simulink model "proof_of_concept"  (R2026a)
settings: Solver=ode4  StopTime=120  FixedStep=0.002
undefined symbols (not defined in the file or in its folder): IC0
libraries: simulink x1
settings Model: Creator=aayush  LastModifiedBy=aayush

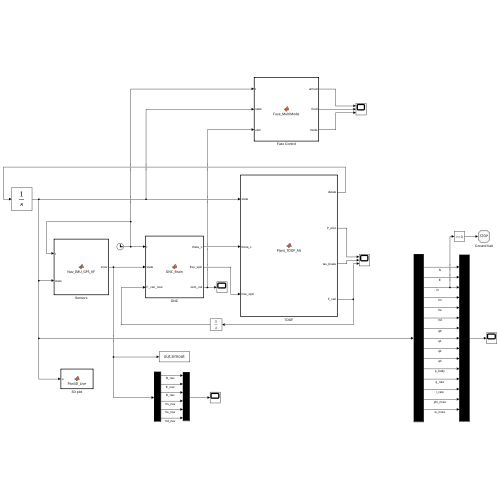
[thumbnail: Simulink's stored preview of the top-level diagram]
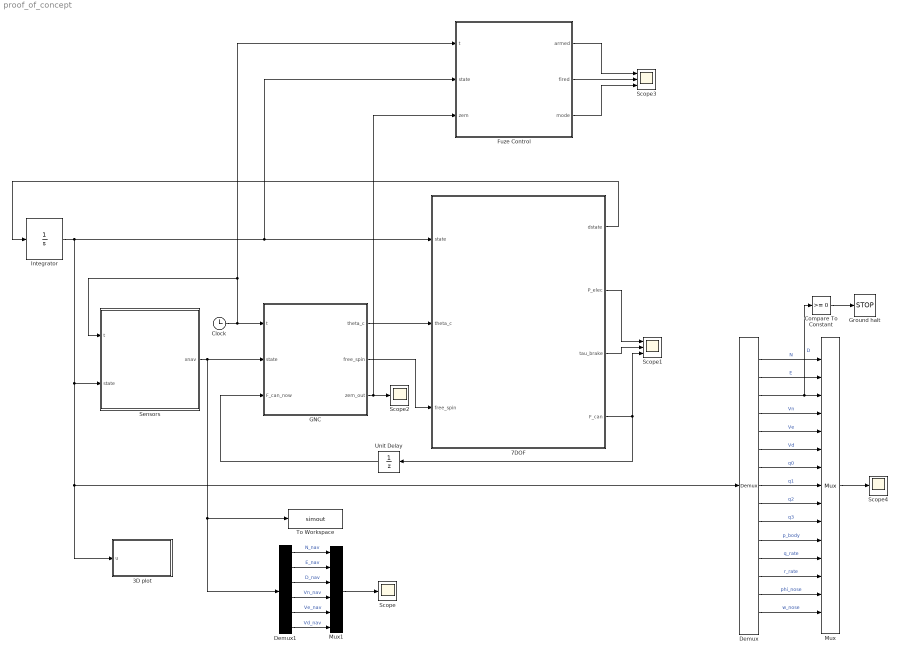
== system proof_of_concept ==
  3D plot : MATLAB Function  TreatAsAtomicUnit=on
  7DOF : MATLAB Function  TreatAsAtomicUnit=on
  Clock : Clock
  Compare To Constant : simulink/Logic and Bit Operations/Compare To Constant  relop=>=  const=0  OutDataTypeStr=boolean
  Demux : Demux  Outputs=15
  Demux1 : Demux  Outputs=6
  Fuze Control : MATLAB Function  TreatAsAtomicUnit=on
  GNC : MATLAB Function  TreatAsAtomicUnit=on
  Ground halt : Stop
  Integrator : Integrator  InitialCondition=IC0
  Mux : Mux  Inputs=15
  Mux1 : Mux  Inputs=6
  Scope : Scope
      settings: ActiveDisplayYMinimum=-6497.6621152905909  ActiveDisplayYMaximum=23835.158611575058
  Scope1 : Scope  NumInputPorts=3
      settings: ActiveDisplayYMinimum=-36.379053196985673  ActiveDisplayYMaximum=247.41147877287113
  Scope2 : Scope
      settings: ActiveDisplayYMinimum=-412.03643421286256  ActiveDisplayYMaximum=3708.3279079157642  DataLoggingVariableName=ScopeData2
  Scope3 : Scope  NumInputPorts=3
      settings: ActiveDisplayYMinimum=-0.12499999999999997  ActiveDisplayYMaximum=1.125  DataLoggingVariableName=ScopeData3
  Scope4 : Scope
      settings: ActiveDisplayYMinimum=-6498.1534286877359  ActiveDisplayYMaximum=23841.089492594823  DataLoggingVariableName=ScopeData4
  Sensors : MATLAB Function  TreatAsAtomicUnit=on
  To Workspace : ToWorkspace  VariableName=simout  SaveFormat=Timeseries  SampleTime=-1
  Unit Delay : UnitDelay  SampleTime=-1
  wires:
  GNC/1(theta_c) -> 7DOF/2(theta_c)
  GNC/2(free_spin) -> 7DOF/3(free_spin)
  7DOF/1(dstate) -> Integrator/1
  Clock/1 -> GNC/1(t), Fuze Control/1(t), Sensors/1(t)
  Integrator/1 -> Demux/1, 3D plot/1(u), Sensors/2(state), Fuze Control/2(state), 7DOF/1(state)
  7DOF/3(tau_brake) -> Scope1/2
  7DOF/2(P_elec) -> Scope1/1
  7DOF/4(F_can) -> Unit Delay/1, Scope1/3
  GNC/3(zem_out) -> Fuze Control/3(zem), Scope2/1
  Unit Delay/1 -> GNC/3(F_can_now)
  Sensors/1(xnav) -> Demux1/1, To Workspace/1, GNC/2(state)
  Fuze Control/2(fired) -> Scope3/2
  Fuze Control/1(armed) -> Scope3/1
  Fuze Control/3(mode) -> Scope3/3
  Demux/1 -> Mux/1  "N"
  Demux/2 -> Mux/2  "E"
  Demux/3 -> Compare To Constant/1, Mux/3  "D"
  Demux/4 -> Mux/4  "Vn"
  Demux/5 -> Mux/5  "Ve"
  Demux/6 -> Mux/6  "Vd"
  Demux/7 -> Mux/7  "q0"
  Demux/8 -> Mux/8  "q1"
  Demux/9 -> Mux/9  "q2"
  Demux/10 -> Mux/10  "q3"
  Demux/11 -> Mux/11  "p_body"
  Demux/12 -> Mux/12  "q_rate"
  Demux/13 -> Mux/13  "r_rate"
  Demux/14 -> Mux/14  "phi_nose"
  Demux/15 -> Mux/15  "w_nose"
  Demux1/3 -> Mux1/3  "D_nav"
  Demux1/1 -> Mux1/1  "N_nav"
  Demux1/2 -> Mux1/2  "E_nav"
  Demux1/4 -> Mux1/4  "Vn_nav"
  Demux1/5 -> Mux1/5  "Ve_nav"
  Demux1/6 -> Mux1/6  "Vd_nav"
  Mux1/1 -> Scope/1
  Mux/1 -> Scope4/1
  Compare To Constant/1 -> Ground halt/1

== matlab function proof_of_concept/GNC ==
  settings: updateMethod=DISCRETE
  data: t input; theta_c output; state input; free_spin output; zem_out output; F_can_now input
function [theta_c, free_spin, zem_out] = GNC_Brain(t, state, F_can_now)
    persistent th_c fs last_F tgt_xy locked mode_free checked failsafe next_ctrl zem_p
    if isempty(th_c) || t < 0.05
        th_c = 0; fs = true; last_F = 0; tgt_xy = [0;0];
        locked = false; mode_free = true; checked = false;
        failsafe = false; next_ctrl = 0; zem_p = 0;
    end
    last_F = 0.65*last_F + 0.35*F_can_now;
    theta_c = th_c; free_spin = fs; zem_out = zem_p;
    if t < next_ctrl, return; end
    next_ctrl = t + 0.02;

    Om_E  = 7.292115e-5*[cos(32*pi/180); 0; -sin(32*pi/180)];
    Mg    = [0.5 0.8 0.95 1.05 1.2 1.5 2.0 2.5];
    Cdrow = [0.13 0.145 0.24 0.30 0.255 0.20 0.18 0.17];

    r = state(1:3); v = state(4:6);
    sp0 = norm(v); if sp0 < 1.0, sp0 = 1.0; end
    vhat0 = v/sp0;
    des = [cos(th_c); sin(th_c); 0];
    fd = des - dot(des,vhat0)*vhat0;
    nfd = norm(fd); if nfd > 1e-6, fd = fd/nfd; else fd = [0;0;0]; end
    F_vec = last_F * fd;

    rr = r; vv = v; tp = 0;
    while rr(3) < 0 && tp < 70
        sp = norm(vv); if sp < 1.0, sp = 1.0; end
        h = max(-rr(3), 0);
        T = max(288.15 - 0.0065*h, 210.0);
        rho = 1.225*(T/288.15)^4.2559;
        Cd0 = lut(sp/sqrt(1.4*287.05*T), Mg, Cdrow);
        a = -Cd0*(0.5*rho*sp^2)*0.01887/43.5*(vv/sp) + F_vec/43.5 ...
            + [0;0;9.80665*(6371000/(6371000+h))^2] - 2*cross(Om_E, vv);
        vv = vv + a*0.1;
        rr = rr + vv*0.1;
        tp = tp + 0.1;
    end

    arm_time = 7.0; deadband = 0.0;    % PoC: hold to impact (no coast switch)
    if ~locked && t >= arm_time
        imp0 = predict0(r, v);
        tgt_xy = imp0(1:2) + [100; -70];
        locked = true;
    end

    if t < arm_time || failsafe
        fs = true; zem_p = 0;
    else
        zem_vec = tgt_xy - rr(1:2);
        zem = norm(zem_vec);
        zem_p = zem; zem_out = zem;
        if ~checked && t >= 8.0
            checked = true;
            if zem > 20000.0, failsafe = true; end
        end
        if ~failsafe
            if mode_free
                if zem >= 1.5*deadband, mode_free = false; end
            else
                if zem < deadband, mode_free = true; end
            end
        end
        fs = mode_free || failsafe;
        if ~fs
            desired = atan2(zem_vec(2), zem_vec(1));
            err = wrapPi(desired - th_c);
            rate = max(min(6.0*err, 1.5708), -1.5708);
            th_c = th_c + (0.02/(0.25+0.02))*rate*0.25;
        end
    end
    theta_c = th_c; free_spin = fs;
end

function imp = predict0(r, v)
    Om_E  = 7.292115e-5*[cos(32*pi/180); 0; -sin(32*pi/180)];
    Mg    = [0.5 0.8 0.95 1.05 1.2 1.5 2.0 2.5];
    Cdrow = [0.13 0.145 0.24 0.30 0.255 0.20 0.18 0.17];
    rr = r; vv = v; tp = 0;
    while rr(3) < 0 && tp < 70
        sp = norm(vv); if sp < 1.0, sp = 1.0; end
        h = max(-rr(3), 0);
        T = max(288.15 - 0.0065*h, 210.0);
        rho = 1.225*(T/288.15)^4.2559;
        Cd0 = lut(sp/sqrt(1.4*287.05*T), Mg, Cdrow);
        a = -Cd0*(0.5*rho*sp^2)*0.01887/43.5*(vv/sp) ...
            + [0;0;9.80665*(6371000/(6371000+h))^2] - 2*cross(Om_E, vv);
        vv = vv + a*0.1;
        rr = rr + vv*0.1;
        tp = tp + 0.1;
    end
    imp = [rr(1); rr(2); 0];
end

function y = lut(M, Mg, Vg)
    n = numel(Mg);
    if M <= Mg(1), y = Vg(1); return; end
    if M >= Mg(n), y = Vg(n); return; end
    k = 1;
    while k < n-1 && M > Mg(k+1), k = k+1; end
    y = Vg(k) + (M-Mg(k))/(Mg(k+1)-Mg(k)) * (Vg(k+1)-Vg(k));
end
function y = wrapPi(x)
    y = mod(x + pi, 2*pi) - pi;
end

== matlab function proof_of_concept/7DOF ==
  data: state input; dstate output; theta_c input; free_spin input; P_elec output; tau_brake output; F_can output
function [dstate, P_elec, tau_brake, F_can] = Plant_7DOF_Alt(state, theta_c, free_spin)
    r = state(1:3); v = state(4:6); q = state(7:10);
    w_b = state(11:13); phi_n = state(14); w_n = state(15);

    m = 43.5; Ixx = 0.148; Iyy = 1.82; Izz = 1.82; Ixx_n = 0.012;
    S = 0.01887; d = 0.155; r_c = 0.48;
    lat = 32*pi/180; Re = 6371000;
    Om_E = 7.292115e-5*[cos(lat); 0; -sin(lat)];

    h = max(-r(3), 0);
    T = max(288.15 - 0.0065*h, 210.0);
    rho = 1.225*(T/288.15)^4.2559;
    a_snd = sqrt(1.4*287.05*T);
    g_mag = 9.80665*(Re/(Re+h))^2;

    speed = norm(v); if speed < 1.0, speed = 1.0; end
    vhat = v/speed;
    M = speed/a_snd;
    qdyn = 0.5*rho*speed^2;

    % ===== Aero LUT (calibrated row; IDENTICAL in GNC predictors) =====
    Mg = [0.5 0.8 0.95 1.05 1.2 1.5 2.0 2.5];
    Cd0  = lut(M, Mg, [0.13 0.145 0.24 0.30 0.255 0.20 0.18 0.17]);
    Cl_a = lut(M, Mg, [1.70 1.68 1.55 1.45 1.50 1.55 1.50 1.45]);
    Cm_a = lut(M, Mg, [-2.4 -2.35 -2.1 -1.95 -2.15 -2.3 -2.25 -2.2]);
    Clp  = lut(M, Mg, [-0.04 -0.042 -0.05 -0.055 -0.05 -0.048 -0.045 -0.043]);
    Cmq  = lut(M, Mg, [-3.8 -4.0 -4.5 -4.6 -4.3 -4.1 -4.0 -3.9]);
    Cn_pa= lut(M, Mg, [0.04 0.05 0.07 0.08 0.06 0.05 0.04 0.035]);
    Cm_pa= lut(M, Mg, [-0.003 -0.0035 -0.005 -0.0055 -0.0045 -0.004 -0.0035 -0.003]);

    R = q_to_dcm(q); body_x = R(:,1);
    ca = max(min(dot(body_x, vhat),1),-1); aoa = acos(ca);
    F_drag = -Cd0*qdyn*S*vhat;
    F_lift = [0;0;0]; F_mag = [0;0;0]; M_im = [0;0;0];
    if aoa > 1e-4 && speed > 35
        ldir = (body_x - ca*vhat); ldir = ldir/norm(ldir);
        if free_spin
            Cl = 0.0;                              % rotating canards: net lift = 0
        else
            Cl = max(min(Cl_a*aoa, 1.05), -1.05);  % maneuvering: follow LUT
        end
        F_lift = Cl*qdyn*S*ldir;
        F_drag = F_drag - (Cl^2/(pi*0.75*5.2))*qdyn*S*vhat;
        axis2 = cross(body_x, vhat); axis2 = axis2/norm(axis2);
        pbar = w_b(1)*d/(2*speed);
        M_im = (-Cm_a*qdyn*S*d*aoa)*axis2 + (Cm_pa*qdyn*S*d*pbar*aoa)*axis2;
        F_mag = (Cn_pa*qdyn*S*pbar*aoa)*axis2;
    end

    % ===== Canards (hold/maneuver only, 3-D perpendicular force) =====
    F_can = [0;0;0];
    if ~free_spin && speed > 70 && abs(w_n) < 40
        CN0 = 1.0*0.68*0.00075/S;
        a_deg = aoa*180/pi;
        f_alpha = max(min(0.88 + 0.012*a_deg - 0.00015*a_deg^2, 1.25), 0.85);
        if aoa >= 0.95*(16*pi/180), f_alpha = f_alpha*0.7; end
        if M < 0.7, f_mach = 1.0;
        elseif M < 1.1, f_mach = 1.0 - 0.15*(M-0.7)/0.4;
        else, f_mach = 0.82; end
        f_mach = max(min(f_mach, 1.05), 0.75);
        f_spin = max(min(1.0 - (w_n/40.0)^2, 1.0), 0.0);
        cy = CN0*f_alpha*f_mach*f_spin;
        Fmag = min(cy*qdyn*S, 1.05*m);
        desired = [cos(phi_n); sin(phi_n); 0];
        f_dir = desired - dot(desired, vhat)*vhat;
        nrm = norm(f_dir);
        if nrm > 1e-6
            F_can = (Fmag/nrm)*f_dir;
            F_lift = F_lift*(1.0 - 0.15*min(Fmag/(qdyn*S), 1.0));
            F_drag = F_drag - 0.05*(Fmag/(qdyn*S))^2*qdyn*S*vhat;
        end
    end
    F_total = F_drag + F_lift + F_can + F_mag;

    kd = qdyn*S*d*(d/(2*speed));
    M_damp = [Clp*kd*w_b(1); Cmq*kd*w_b(2); Cmq*kd*w_b(3)];
    M_can = cross([r_c;0;0], R'*F_can);
    M_body = M_can + M_damp + R'*M_im;

    % ===== Dual-spin brake + alternator =====
    w_rel = w_n - w_b(1);
    tau_aero = 0.0;
    if speed > 40
        tau_aero = -0.00040*qdyn*sign(w_n)*min(abs(w_n)/80.0, 1.0);
        if abs(w_n) < 6.0, tau_aero = tau_aero*0.2; end
    end
    tau_alt = -0.00025*w_rel;
    if free_spin
        tau_cmd = tau_aero + tau_alt;
    else
        err_phi = wrapPi(theta_c - phi_n);
        tau_cmd = 0.15*tau_aero + tau_alt - 1.0*w_n + 30.0*err_phi;
    end
    tau_brake = max(min(tau_cmd, 8.0), -8.0) - 0.0015*w_rel;
    M_body(1) = M_body(1) - tau_brake;

    P_elec = 0.65*(1 - exp(-abs(w_rel)/200))*abs(tau_alt*w_rel);

    wdot = [ (M_body(1) - (Iyy-Izz)*w_b(2)*w_b(3))/Ixx;
             (M_body(2) - (Izz-Ixx)*w_b(3)*w_b(1))/Iyy;
             (M_body(3) - (Ixx-Iyy)*w_b(1)*w_b(2))/Izz ];

    dstate = zeros(15,1);
    dstate(1:3) = v;
    dstate(4:6) = F_total/m + [0;0;g_mag] - 2*cross(Om_E, v);
    dstate(7:10) = q_omega_mult(q, w_b);
    dstate(11:13) = wdot;
    dstate(14) = w_n;
    dstate(15) = tau_brake/Ixx_n;
    F_can = norm(F_can);
end

function y = lut(M, Mg, Vg)
    n = numel(Mg);
    if M <= Mg(1), y = Vg(1); return; end
    if M >= Mg(n), y = Vg(n); return; end
    k = 1;
    while k < n-1 && M > Mg(k+1), k = k+1; end
    y = Vg(k) + (M-Mg(k))/(Mg(k+1)-Mg(k)) * (Vg(k+1)-Vg(k));
end
function R = q_to_dcm(q)
    w=q(1); x=q(2); y=q(3); z=q(4);
    R = [1-2*(y^2+z^2), 2*(x*y-w*z), 2*(x*z+w*y);
         2*(x*y+w*z), 1-2*(x^2+z^2), 2*(y*z-w*x);
         2*(x*z-w*y), 2*(y*z+w*x), 1-2*(x^2+y^2)];
end
function dq = q_omega_mult(q, w)
    p=w(1); qr=w(2); r=w(3);
    Om = [0,-p,-qr,-r; p,0,r,-qr; qr,-r,0,p; r,qr,-p,0];
    dq = 0.5*Om*q;
end
function y = wrapPi(x)
    y = mod(x + pi, 2*pi) - pi;
end

== matlab function proof_of_concept/Sensors ==
  settings: updateMethod=DISCRETE
  data: t input; xnav output; state input
function xnav = Nav_IMU_GPS_KF(t, state)
    persistent x P fix_buf fix_time last_gps_t prev_t v_prev
    N_FIX = 10;
    if isempty(x)
        x = zeros(9,1); P = zeros(9,9);
        fix_buf = zeros(N_FIX,7);
        fix_time = -1e6*ones(1,N_FIX);
        last_gps_t = 0; prev_t = 0; v_prev = zeros(3,1);
    end
    if t < 0.01
        x(1:3) = state(1:3); x(4:6) = state(4:6); x(7:9) = zeros(3,1);
        P = diag([25 25 40 4 4 4 0.01 0.01 0.01]);
        fix_buf = zeros(N_FIX,7);
        fix_time = -1e6*ones(1,N_FIX);
        last_gps_t = 0; prev_t = 0; v_prev = state(4:6);
    end
    dt = t - prev_t;
    if dt < 0, dt = 0; end
    if dt > 0.02, dt = 0.02; end
    prev_t = t;

    % ===== IMU (200 Hz): specific force from velocity difference =====
    g_vec = [0; 0; 9.80665];
    if dt > 0
        a_tot = (state(4:6) - v_prev)/dt;
    else
        a_tot = zeros(3,1);
    end
    v_prev = state(4:6);
    a_truth = a_tot - g_vec;
    a_meas = a_truth + x(7:9) + 0.08*randn(3,1);

    % ===== Predict (strapdown, gravity restored) =====
    x(1:3) = x(1:3) + x(4:6)*dt;
    x(4:6) = x(4:6) + (a_meas - x(7:9) + g_vec)*dt;
    x(7:9) = x(7:9) + 5e-5*randn(3,1);
    F = eye(9);
    F(1:3,4:6) = eye(3)*dt;
    F(4:6,7:9) = -eye(3)*dt;
    Q = diag([0 0 0 0.5*dt 0.5*dt 0.5*dt 1e-5 1e-5 1e-5]);
    P = F*P*F' + Q;

    % ===== GPS fix generation (50 Hz) =====
    if t - last_gps_t >= 0.019
        last_gps_t = t;
        z_pos = state(1:3) + [2.5; 2.5; 3.75].*randn(3,1);
        z_vel = state(4:6) + 0.25*randn(3,1);
        idx = mod(round(t/0.02), N_FIX) + 1;
        fix_buf(idx,:) = [t, z_pos(1), z_pos(2), z_pos(3), ...
                             z_vel(1), z_vel(2), z_vel(3)];
        fix_time(idx) = t;
    end

    % ===== Apply fixes with 20 ms latency =====
    for i = 1:N_FIX
        if fix_time(i) > -1e5 && fix_time(i) <= t - 0.02
            zp = fix_buf(i,2:4)';
            zv = fix_buf(i,5:7)';
            fix_time(i) = -1e6;
            Hp = [eye(3) zeros(3,6)];
            Rp = diag([6.25 6.25 14.0625]);
            yp = zp - Hp*x;
            Sp = Hp*P*Hp' + Rp;
            Kp = P*Hp'/Sp;
            x = x + Kp*yp;
            P = (eye(9) - Kp*Hp)*P;
            Hv = [zeros(3,3) eye(3) zeros(3,3)];
            Rv = 0.0625*eye(3);
            yv = zv - Hv*x;
            Sv = Hv*P*Hv' + Rv;
            Kv = P*Hv'/Sv;
            x = x + Kv*yv;
            P = (eye(9) - Kv*Hv)*P;
        end
    end
    xnav = x(1:6);
end

== matlab function proof_of_concept/Fuze Control ==
  settings: updateMethod=DISCRETE
  data: t input; armed output; state input; zem input; fired output; mode output
function [armed, fired, mode] = Fuze_MultiMode(t, state, zem)
    persistent t0 inhibit checked
    if isempty(t0) || t < 0.05
        t0 = -1.0; inhibit = false; checked = false;
    end
    h = -state(3);
    if t0 < 0 && t > 0.05
        t0 = t;
    end
    safe_delay = 0.8;
    mode_sel   = 0;        % 0=IMPACT, 1=TIME, 2=PROXIMITY
    time_func  = 25.0;
    prox_h     = 10.0;
    if ~checked && t0 > 0 && (t - t0) >= 5.0
        checked = true;
        if zem > 150.0
            inhibit = true;
        end
    end
    armed = (t0 > 0) && ((t - t0) >= safe_delay) && ~inhibit;
    fired = false;
    if armed
        if mode_sel == 0
            fired = (h <= 0.0);
        elseif mode_sel == 1
            fired = ((t - t0) >= time_func);
        else
            fired = (h <= prox_h && (t - t0) > safe_delay + 1.0) || (h <= 0.0);
        end
    end
    mode = mode_sel;
end

== matlab function proof_of_concept/3D plot ==
  settings: updateMethod=DISCRETE
  data: u input
function Plot3D_Live(u)
coder.extrinsic('live3d');
live3d(u);
end
